simulink model "Q5_2_2"  (R2023b)
settings: Solver=ode45  StartTime=0.0  StopTime=15.0  FixedStep=0.001  RelTol=1e-3
settings Model: Creator=Arshia  LastModifiedBy=Arshia

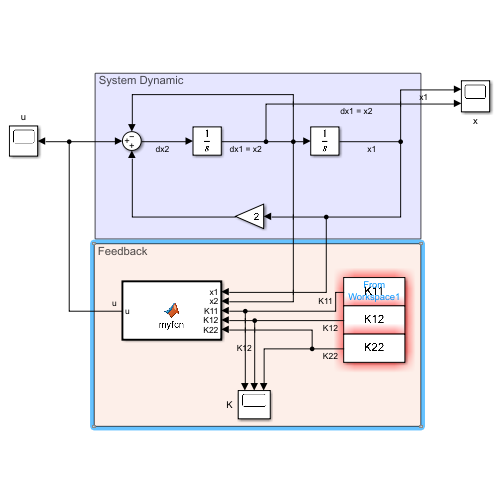
[thumbnail: Simulink's stored preview of the top-level diagram]
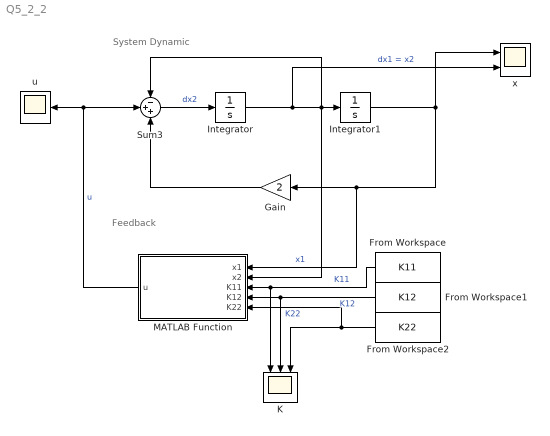
== system Q5_2_2 ==
  note: Feedback
  note: System Dynamic
  From Workspace : FromWorkspace  VariableName=K11
  From Workspace1 : FromWorkspace  VariableName=K12
  From Workspace2 : FromWorkspace  VariableName=K22
  Gain : Gain  Gain=2
  Integrator : Integrator  InitialCondition=4
  Integrator1 : Integrator  InitialCondition=-4
  K : Scope  NumInputPorts=3
  MATLAB Function : MATLAB Function  TreatAsAtomicUnit=on
  Sum3 : Sum  Inputs=-++
  u : Scope
  x : Scope  NumInputPorts=2
  wires:
  Gain/1 -> Sum3/3
  Integrator/1 -> x/2, Sum3/1, MATLAB Function/2(x2), Integrator1/1  "dx1 = x2"
  Sum3/1 -> Integrator/1  "dx2"
  Integrator1/1 -> MATLAB Function/1(x1), Gain/1, x/1  "x1"
  MATLAB Function/1(u) -> Sum3/2, u/1  "u"
  From Workspace/1 -> MATLAB Function/3(K11), K/1  "K11"
  From Workspace1/1 -> K/2, MATLAB Function/4(K12)  "K12"
  From Workspace2/1 -> MATLAB Function/5(K22), K/3  "K22"

== matlab function Q5_2_2/MATLAB Function ==
  data: u output; x1 input; x2 input; K11 input; K12 input; K22 input
function u =myfcn(x1,x2,K11,K12,K22)
R=1/2;
B=[0 1]';
x=[x1 x2]';
u=-(R)^-1*B'*[K11 K12;K12 K22]*x;
end
